simulink model "DWPT_250k_60V"  (R2026b)
settings: Solver=ode3  StopTime=0.03  FixedStep=Ts  MaxStep=1.0E-7  RelTol=1e-4  AbsTol=1e-6
model workspace (MAT data in the model file):
  CP1 = 9.99954859124e-09
  CS = 8.10569469139e-09
  CT1 = 4.27980679705e-08
  Cout = 0.00047
  Goff = 1e-08
  Ki = 20
  Kp = 0.015
  LP1 = 5e-05
  LS = 5e-05
  LT1 = 9.4696969697e-06
  M1 = 1.25e-05
  Mdesign = 1.25e-05
  RL = 30
  RP1 = 0.2
  RS = 0.2
  RT1 = 0.07
  RonSR = 0.01
  RonTx = 0.01
  Ts = 1e-08
  Vavailable = 66
  Vdc = 50
  Vtarget = 60
  averageCycles = 100
  bodyRon = 0.01
  bodyVf = 0.8
  closedLoop = 1
  deadTime = 4e-08
  f = 250000
  initialOutputVoltage = 0
  k = 0.25
  samplesPerPeriod = 400
  softStart = 0.02
  srDeadTime = 4e-08
  srEnabled = 1
  srThreshold = 0.1
  voltageHeadroom = 1.1
undefined symbols (not defined in the file or in its folder): ee_sli_rtmsupport, G, gcbh
libraries: sl_signal_attributes x63, eeGeneralControl x37, fl_lib x32, nesl_utility x28, eeGeneralMeasurement x14, ee_lib x8, dspfdesign x1
(part 2 of 3)

== system DWPT_250k_60V/Product1 ==
  Current : Inport
  Voltage : Inport  Port=2
  Average power : eeGeneralControl/Moving Average  VariantControl=Variant1  LabelModeActiveChoice=Continuous  f=f/averageCycles  x0=0  BufferSize=8192  Ts=0
      link override Continuous/Transport Delay: BufferSize=262144
  Instantaneous power : Product
  Watts : Outport
  wires:
  Current/1 -> Instantaneous power/1
  Voltage/1 -> Instantaneous power/2
  Instantaneous power/1 -> Average power/1
  Average power/1 -> Watts/1

== system DWPT_250k_60V/Product4 ==
  Current : Inport
  Voltage : Inport  Port=2
  Average power : eeGeneralControl/Moving Average  VariantControl=Variant1  LabelModeActiveChoice=Continuous  f=f/averageCycles  x0=0  BufferSize=8192  Ts=0
      link override Continuous/Transport Delay: BufferSize=262144
  Instantaneous power : Product
  Watts : Outport
  wires:
  Current/1 -> Instantaneous power/1
  Voltage/1 -> Instantaneous power/2
  Instantaneous power/1 -> Average power/1
  Average power/1 -> Watts/1

== system DWPT_250k_60V/R4 ==
  Resistor : fl_lib/Electrical/Electrical Elements/Resistor  R=RL Ohm  i_specify=off  i_priority=None  i=0 A  i_nominal_specify=off  i_nominal_value=1  i_nominal_unit=A  v_specify=off  v_priority=None  v=0 V  v_nominal_specify=off  v_nominal_value=1  v_nominal_unit=V
  + : PMIOPort  Side=Left
  - : PMIOPort  Port=2  Side=Right
  connections:
  +/RConn1 -- Resistor/LConn1
  -/RConn1 -- Resistor/RConn1

== system DWPT_250k_60V/RMS1 ==
  In : Inport
  RMS Measurement : Subsystem  LoadFcn=ee_sli_rtmsupport( 'loadfcn', gcbh );  Variant=on  VariantControlMode=label  LabelModeActiveChoice=Total  mask(RMS Measurement){F=f/averageCycles, SpecifyHarmonics=off, K=[0 1 2], InitialRMS=0, Ts=0}
      mask prompts: F "physmod:ee:library:comments:control:eeRmsMeasurement:BaseFrequencyHz_MP"; SpecifyHarmonics "physmod:ee:library:comments:control:eeRmsMeasurement:SpecifyHarmonics_MP"; K "physmod:ee:library:comments:control:eeRmsMeasurement:HarmonicNumbers_MP"; InitialRMS "physmod:ee:library:comments:control:eeRmsMeasurement:InitialRMS_MP"; Ts "physmod:ee:library:comments:control:eeGeneralControl:SampleTime1ForInherited_MP"
      mask help: physmod:ee:library:comments:control:eeRmsMeasurement:RMSMeasurement_MD
      mask init:
      | [timeDomain,G]=ee.mask.initializeRmsMeasurement(gcb,F,Ts,K,SpecifyHarmonics,InitialRMS);
      settings: CopyFcn=ee_sli_rtmsupport( 'copyfcn', gcbh );  DeleteFcn=ee_sli_rtmsupport( 'deletefcn', gcbh );  ModelCloseFcn=ee_sli_rtmsupport( 'modelclosefcn', gcbh );  PostSaveFcn=ee_sli_rtmsupport( 'postsavefcn', gcbh );  PreCopyFcn=ee_sli_rtmsupport( 'precopyfcn', gcbh );  OpenFcn=ee_sli_rtmsupport( 'openfcn', gcbh );  CloseFcn=ee_sli_rtmsupport( 'closefcn', gcbh );  PreDeleteFcn=ee_sli_rtmsupport( 'predeletefcn', gcbh );
      mask Help: web(nesl_help(gcbh))
      mask Callback SpecifyHarmonics: ee.mask.callbackRmsMeasurement(gcb);
      mask TypeOptions Ts:
      | Total RMS/Integrator
      | (Discrete or Continuous)/Ts | Total RMS/Integrator
      | (Discrete or Continuous)1/Ts | Total RMS/Periodic Difference
      | (Discrete or Continuous)/Ts | Harmonic RMS/Integrator
      | (Discrete or Continuous)/Ts | Harmonic RMS/Integrator
      | (Discrete or Continuous)1/Ts | Harmonic RMS/Periodic Difference
      | (Discrete or Continuous)/Ts | Harmonic RMS/SinCos/Integrator with
      | Wrapped State
      | (Discrete or Continuous)/Ts
      mask DialogControl F Prompt: Base frequency (Hz)
      mask DialogControl SpecifyHarmonics Prompt: Specify harmonics
      mask DialogControl K Prompt: Harmonic numbers
      mask DialogControl InitialRMS Prompt: Initial RMS
      mask DialogControl Ts Prompt: Sample time (-1 for inherited)
      mask Display: ee.mask.drawRmsMeasurement;
  RMS : Outport  VectorParamsAs1DForOutWhenUnconnected=off
  wires:
  RMS Measurement/1(RMS) -> RMS/1
  In/1 -> RMS Measurement/1(u)

== system DWPT_250k_60V/RMS10 ==
  In : Inport
  RMS Measurement : Subsystem  LoadFcn=ee_sli_rtmsupport( 'loadfcn', gcbh );  Variant=on  VariantControlMode=label  LabelModeActiveChoice=Total  mask(RMS Measurement){F=f/averageCycles, SpecifyHarmonics=off, K=[0 1 2], InitialRMS=0, Ts=0}
      mask prompts: F "physmod:ee:library:comments:control:eeRmsMeasurement:BaseFrequencyHz_MP"; SpecifyHarmonics "physmod:ee:library:comments:control:eeRmsMeasurement:SpecifyHarmonics_MP"; K "physmod:ee:library:comments:control:eeRmsMeasurement:HarmonicNumbers_MP"; InitialRMS "physmod:ee:library:comments:control:eeRmsMeasurement:InitialRMS_MP"; Ts "physmod:ee:library:comments:control:eeGeneralControl:SampleTime1ForInherited_MP"
      mask help: physmod:ee:library:comments:control:eeRmsMeasurement:RMSMeasurement_MD
      mask init:
      | [timeDomain,G]=ee.mask.initializeRmsMeasurement(gcb,F,Ts,K,SpecifyHarmonics,InitialRMS);
      settings: CopyFcn=ee_sli_rtmsupport( 'copyfcn', gcbh );  DeleteFcn=ee_sli_rtmsupport( 'deletefcn', gcbh );  ModelCloseFcn=ee_sli_rtmsupport( 'modelclosefcn', gcbh );  PostSaveFcn=ee_sli_rtmsupport( 'postsavefcn', gcbh );  PreCopyFcn=ee_sli_rtmsupport( 'precopyfcn', gcbh );  OpenFcn=ee_sli_rtmsupport( 'openfcn', gcbh );  CloseFcn=ee_sli_rtmsupport( 'closefcn', gcbh );  PreDeleteFcn=ee_sli_rtmsupport( 'predeletefcn', gcbh );
      mask Help: web(nesl_help(gcbh))
      mask Callback SpecifyHarmonics: ee.mask.callbackRmsMeasurement(gcb);
      mask TypeOptions Ts:
      | Total RMS/Integrator
      | (Discrete or Continuous)/Ts | Total RMS/Integrator
      | (Discrete or Continuous)1/Ts | Total RMS/Periodic Difference
      | (Discrete or Continuous)/Ts | Harmonic RMS/Integrator
      | (Discrete or Continuous)/Ts | Harmonic RMS/Integrator
      | (Discrete or Continuous)1/Ts | Harmonic RMS/Periodic Difference
      | (Discrete or Continuous)/Ts | Harmonic RMS/SinCos/Integrator with
      | Wrapped State
      | (Discrete or Continuous)/Ts
      mask DialogControl F Prompt: Base frequency (Hz)
      mask DialogControl SpecifyHarmonics Prompt: Specify harmonics
      mask DialogControl K Prompt: Harmonic numbers
      mask DialogControl InitialRMS Prompt: Initial RMS
      mask DialogControl Ts Prompt: Sample time (-1 for inherited)
      mask Display: ee.mask.drawRmsMeasurement;
  RMS : Outport  VectorParamsAs1DForOutWhenUnconnected=off
  wires:
  RMS Measurement/1(RMS) -> RMS/1
  In/1 -> RMS Measurement/1(u)

== system DWPT_250k_60V/RMS2 ==
  In : Inport
  RMS Measurement : Subsystem  LoadFcn=ee_sli_rtmsupport( 'loadfcn', gcbh );  Variant=on  VariantControlMode=label  LabelModeActiveChoice=Total  mask(RMS Measurement){F=f/averageCycles, SpecifyHarmonics=off, K=[0 1 2], InitialRMS=0, Ts=0}
      mask prompts: F "physmod:ee:library:comments:control:eeRmsMeasurement:BaseFrequencyHz_MP"; SpecifyHarmonics "physmod:ee:library:comments:control:eeRmsMeasurement:SpecifyHarmonics_MP"; K "physmod:ee:library:comments:control:eeRmsMeasurement:HarmonicNumbers_MP"; InitialRMS "physmod:ee:library:comments:control:eeRmsMeasurement:InitialRMS_MP"; Ts "physmod:ee:library:comments:control:eeGeneralControl:SampleTime1ForInherited_MP"
      mask help: physmod:ee:library:comments:control:eeRmsMeasurement:RMSMeasurement_MD
      mask init:
      | [timeDomain,G]=ee.mask.initializeRmsMeasurement(gcb,F,Ts,K,SpecifyHarmonics,InitialRMS);
      settings: CopyFcn=ee_sli_rtmsupport( 'copyfcn', gcbh );  DeleteFcn=ee_sli_rtmsupport( 'deletefcn', gcbh );  ModelCloseFcn=ee_sli_rtmsupport( 'modelclosefcn', gcbh );  PostSaveFcn=ee_sli_rtmsupport( 'postsavefcn', gcbh );  PreCopyFcn=ee_sli_rtmsupport( 'precopyfcn', gcbh );  OpenFcn=ee_sli_rtmsupport( 'openfcn', gcbh );  CloseFcn=ee_sli_rtmsupport( 'closefcn', gcbh );  PreDeleteFcn=ee_sli_rtmsupport( 'predeletefcn', gcbh );
      mask Help: web(nesl_help(gcbh))
      mask Callback SpecifyHarmonics: ee.mask.callbackRmsMeasurement(gcb);
      mask TypeOptions Ts:
      | Total RMS/Integrator
      | (Discrete or Continuous)/Ts | Total RMS/Integrator
      | (Discrete or Continuous)1/Ts | Total RMS/Periodic Difference
      | (Discrete or Continuous)/Ts | Harmonic RMS/Integrator
      | (Discrete or Continuous)/Ts | Harmonic RMS/Integrator
      | (Discrete or Continuous)1/Ts | Harmonic RMS/Periodic Difference
      | (Discrete or Continuous)/Ts | Harmonic RMS/SinCos/Integrator with
      | Wrapped State
      | (Discrete or Continuous)/Ts
      mask DialogControl F Prompt: Base frequency (Hz)
      mask DialogControl SpecifyHarmonics Prompt: Specify harmonics
      mask DialogControl K Prompt: Harmonic numbers
      mask DialogControl InitialRMS Prompt: Initial RMS
      mask DialogControl Ts Prompt: Sample time (-1 for inherited)
      mask Display: ee.mask.drawRmsMeasurement;
  RMS : Outport  VectorParamsAs1DForOutWhenUnconnected=off
  wires:
  RMS Measurement/1(RMS) -> RMS/1
  In/1 -> RMS Measurement/1(u)

== system DWPT_250k_60V/RMS3 ==
  In : Inport
  RMS Measurement : Subsystem  LoadFcn=ee_sli_rtmsupport( 'loadfcn', gcbh );  Variant=on  VariantControlMode=label  LabelModeActiveChoice=Total  mask(RMS Measurement){F=f/averageCycles, SpecifyHarmonics=off, K=[0 1 2], InitialRMS=0, Ts=0}
      mask prompts: F "physmod:ee:library:comments:control:eeRmsMeasurement:BaseFrequencyHz_MP"; SpecifyHarmonics "physmod:ee:library:comments:control:eeRmsMeasurement:SpecifyHarmonics_MP"; K "physmod:ee:library:comments:control:eeRmsMeasurement:HarmonicNumbers_MP"; InitialRMS "physmod:ee:library:comments:control:eeRmsMeasurement:InitialRMS_MP"; Ts "physmod:ee:library:comments:control:eeGeneralControl:SampleTime1ForInherited_MP"
      mask help: physmod:ee:library:comments:control:eeRmsMeasurement:RMSMeasurement_MD
      mask init:
      | [timeDomain,G]=ee.mask.initializeRmsMeasurement(gcb,F,Ts,K,SpecifyHarmonics,InitialRMS);
      settings: CopyFcn=ee_sli_rtmsupport( 'copyfcn', gcbh );  DeleteFcn=ee_sli_rtmsupport( 'deletefcn', gcbh );  ModelCloseFcn=ee_sli_rtmsupport( 'modelclosefcn', gcbh );  PostSaveFcn=ee_sli_rtmsupport( 'postsavefcn', gcbh );  PreCopyFcn=ee_sli_rtmsupport( 'precopyfcn', gcbh );  OpenFcn=ee_sli_rtmsupport( 'openfcn', gcbh );  CloseFcn=ee_sli_rtmsupport( 'closefcn', gcbh );  PreDeleteFcn=ee_sli_rtmsupport( 'predeletefcn', gcbh );
      mask Help: web(nesl_help(gcbh))
      mask Callback SpecifyHarmonics: ee.mask.callbackRmsMeasurement(gcb);
      mask TypeOptions Ts:
      | Total RMS/Integrator
      | (Discrete or Continuous)/Ts | Total RMS/Integrator
      | (Discrete or Continuous)1/Ts | Total RMS/Periodic Difference
      | (Discrete or Continuous)/Ts | Harmonic RMS/Integrator
      | (Discrete or Continuous)/Ts | Harmonic RMS/Integrator
      | (Discrete or Continuous)1/Ts | Harmonic RMS/Periodic Difference
      | (Discrete or Continuous)/Ts | Harmonic RMS/SinCos/Integrator with
      | Wrapped State
      | (Discrete or Continuous)/Ts
      mask DialogControl F Prompt: Base frequency (Hz)
      mask DialogControl SpecifyHarmonics Prompt: Specify harmonics
      mask DialogControl K Prompt: Harmonic numbers
      mask DialogControl InitialRMS Prompt: Initial RMS
      mask DialogControl Ts Prompt: Sample time (-1 for inherited)
      mask Display: ee.mask.drawRmsMeasurement;
  RMS : Outport  VectorParamsAs1DForOutWhenUnconnected=off
  wires:
  RMS Measurement/1(RMS) -> RMS/1
  In/1 -> RMS Measurement/1(u)

== system DWPT_250k_60V/RMS4 ==
  In : Inport
  RMS Measurement : Subsystem  LoadFcn=ee_sli_rtmsupport( 'loadfcn', gcbh );  Variant=on  VariantControlMode=label  LabelModeActiveChoice=Total  mask(RMS Measurement){F=f/averageCycles, SpecifyHarmonics=off, K=[0 1 2], InitialRMS=0, Ts=0}
      mask prompts: F "physmod:ee:library:comments:control:eeRmsMeasurement:BaseFrequencyHz_MP"; SpecifyHarmonics "physmod:ee:library:comments:control:eeRmsMeasurement:SpecifyHarmonics_MP"; K "physmod:ee:library:comments:control:eeRmsMeasurement:HarmonicNumbers_MP"; InitialRMS "physmod:ee:library:comments:control:eeRmsMeasurement:InitialRMS_MP"; Ts "physmod:ee:library:comments:control:eeGeneralControl:SampleTime1ForInherited_MP"
      mask help: physmod:ee:library:comments:control:eeRmsMeasurement:RMSMeasurement_MD
      mask init:
      | [timeDomain,G]=ee.mask.initializeRmsMeasurement(gcb,F,Ts,K,SpecifyHarmonics,InitialRMS);
      settings: CopyFcn=ee_sli_rtmsupport( 'copyfcn', gcbh );  DeleteFcn=ee_sli_rtmsupport( 'deletefcn', gcbh );  ModelCloseFcn=ee_sli_rtmsupport( 'modelclosefcn', gcbh );  PostSaveFcn=ee_sli_rtmsupport( 'postsavefcn', gcbh );  PreCopyFcn=ee_sli_rtmsupport( 'precopyfcn', gcbh );  OpenFcn=ee_sli_rtmsupport( 'openfcn', gcbh );  CloseFcn=ee_sli_rtmsupport( 'closefcn', gcbh );  PreDeleteFcn=ee_sli_rtmsupport( 'predeletefcn', gcbh );
      mask Help: web(nesl_help(gcbh))
      mask Callback SpecifyHarmonics: ee.mask.callbackRmsMeasurement(gcb);
      mask TypeOptions Ts:
      | Total RMS/Integrator
      | (Discrete or Continuous)/Ts | Total RMS/Integrator
      | (Discrete or Continuous)1/Ts | Total RMS/Periodic Difference
      | (Discrete or Continuous)/Ts | Harmonic RMS/Integrator
      | (Discrete or Continuous)/Ts | Harmonic RMS/Integrator
      | (Discrete or Continuous)1/Ts | Harmonic RMS/Periodic Difference
      | (Discrete or Continuous)/Ts | Harmonic RMS/SinCos/Integrator with
      | Wrapped State
      | (Discrete or Continuous)/Ts
      mask DialogControl F Prompt: Base frequency (Hz)
      mask DialogControl SpecifyHarmonics Prompt: Specify harmonics
      mask DialogControl K Prompt: Harmonic numbers
      mask DialogControl InitialRMS Prompt: Initial RMS
      mask DialogControl Ts Prompt: Sample time (-1 for inherited)
      mask Display: ee.mask.drawRmsMeasurement;
  RMS : Outport  VectorParamsAs1DForOutWhenUnconnected=off
  wires:
  RMS Measurement/1(RMS) -> RMS/1
  In/1 -> RMS Measurement/1(u)

== system DWPT_250k_60V/RMS6 ==
  In : Inport
  RMS Measurement : Subsystem  LoadFcn=ee_sli_rtmsupport( 'loadfcn', gcbh );  Variant=on  VariantControlMode=label  LabelModeActiveChoice=Total  mask(RMS Measurement){F=f/averageCycles, SpecifyHarmonics=off, K=[0 1 2], InitialRMS=0, Ts=0}
      mask prompts: F "physmod:ee:library:comments:control:eeRmsMeasurement:BaseFrequencyHz_MP"; SpecifyHarmonics "physmod:ee:library:comments:control:eeRmsMeasurement:SpecifyHarmonics_MP"; K "physmod:ee:library:comments:control:eeRmsMeasurement:HarmonicNumbers_MP"; InitialRMS "physmod:ee:library:comments:control:eeRmsMeasurement:InitialRMS_MP"; Ts "physmod:ee:library:comments:control:eeGeneralControl:SampleTime1ForInherited_MP"
      mask help: physmod:ee:library:comments:control:eeRmsMeasurement:RMSMeasurement_MD
      mask init:
      | [timeDomain,G]=ee.mask.initializeRmsMeasurement(gcb,F,Ts,K,SpecifyHarmonics,InitialRMS);
      settings: CopyFcn=ee_sli_rtmsupport( 'copyfcn', gcbh );  DeleteFcn=ee_sli_rtmsupport( 'deletefcn', gcbh );  ModelCloseFcn=ee_sli_rtmsupport( 'modelclosefcn', gcbh );  PostSaveFcn=ee_sli_rtmsupport( 'postsavefcn', gcbh );  PreCopyFcn=ee_sli_rtmsupport( 'precopyfcn', gcbh );  OpenFcn=ee_sli_rtmsupport( 'openfcn', gcbh );  CloseFcn=ee_sli_rtmsupport( 'closefcn', gcbh );  PreDeleteFcn=ee_sli_rtmsupport( 'predeletefcn', gcbh );
      mask Help: web(nesl_help(gcbh))
      mask Callback SpecifyHarmonics: ee.mask.callbackRmsMeasurement(gcb);
      mask TypeOptions Ts:
      | Total RMS/Integrator
      | (Discrete or Continuous)/Ts | Total RMS/Integrator
      | (Discrete or Continuous)1/Ts | Total RMS/Periodic Difference
      | (Discrete or Continuous)/Ts | Harmonic RMS/Integrator
      | (Discrete or Continuous)/Ts | Harmonic RMS/Integrator
      | (Discrete or Continuous)1/Ts | Harmonic RMS/Periodic Difference
      | (Discrete or Continuous)/Ts | Harmonic RMS/SinCos/Integrator with
      | Wrapped State
      | (Discrete or Continuous)/Ts
      mask DialogControl F Prompt: Base frequency (Hz)
      mask DialogControl SpecifyHarmonics Prompt: Specify harmonics
      mask DialogControl K Prompt: Harmonic numbers
      mask DialogControl InitialRMS Prompt: Initial RMS
      mask DialogControl Ts Prompt: Sample time (-1 for inherited)
      mask Display: ee.mask.drawRmsMeasurement;
  RMS : Outport  VectorParamsAs1DForOutWhenUnconnected=off
  wires:
  RMS Measurement/1(RMS) -> RMS/1
  In/1 -> RMS Measurement/1(u)

== system DWPT_250k_60V/RMS8 ==
  In : Inport
  RMS Measurement : Subsystem  LoadFcn=ee_sli_rtmsupport( 'loadfcn', gcbh );  Variant=on  VariantControlMode=label  LabelModeActiveChoice=Total  mask(RMS Measurement){F=f/averageCycles, SpecifyHarmonics=off, K=[0 1 2], InitialRMS=0, Ts=0}
      mask prompts: F "physmod:ee:library:comments:control:eeRmsMeasurement:BaseFrequencyHz_MP"; SpecifyHarmonics "physmod:ee:library:comments:control:eeRmsMeasurement:SpecifyHarmonics_MP"; K "physmod:ee:library:comments:control:eeRmsMeasurement:HarmonicNumbers_MP"; InitialRMS "physmod:ee:library:comments:control:eeRmsMeasurement:InitialRMS_MP"; Ts "physmod:ee:library:comments:control:eeGeneralControl:SampleTime1ForInherited_MP"
      mask help: physmod:ee:library:comments:control:eeRmsMeasurement:RMSMeasurement_MD
      mask init:
      | [timeDomain,G]=ee.mask.initializeRmsMeasurement(gcb,F,Ts,K,SpecifyHarmonics,InitialRMS);
      settings: CopyFcn=ee_sli_rtmsupport( 'copyfcn', gcbh );  DeleteFcn=ee_sli_rtmsupport( 'deletefcn', gcbh );  ModelCloseFcn=ee_sli_rtmsupport( 'modelclosefcn', gcbh );  PostSaveFcn=ee_sli_rtmsupport( 'postsavefcn', gcbh );  PreCopyFcn=ee_sli_rtmsupport( 'precopyfcn', gcbh );  OpenFcn=ee_sli_rtmsupport( 'openfcn', gcbh );  CloseFcn=ee_sli_rtmsupport( 'closefcn', gcbh );  PreDeleteFcn=ee_sli_rtmsupport( 'predeletefcn', gcbh );
      mask Help: web(nesl_help(gcbh))
      mask Callback SpecifyHarmonics: ee.mask.callbackRmsMeasurement(gcb);
      mask TypeOptions Ts:
      | Total RMS/Integrator
      | (Discrete or Continuous)/Ts | Total RMS/Integrator
      | (Discrete or Continuous)1/Ts | Total RMS/Periodic Difference
      | (Discrete or Continuous)/Ts | Harmonic RMS/Integrator
      | (Discrete or Continuous)/Ts | Harmonic RMS/Integrator
      | (Discrete or Continuous)1/Ts | Harmonic RMS/Periodic Difference
      | (Discrete or Continuous)/Ts | Harmonic RMS/SinCos/Integrator with
      | Wrapped State
      | (Discrete or Continuous)/Ts
      mask DialogControl F Prompt: Base frequency (Hz)
      mask DialogControl SpecifyHarmonics Prompt: Specify harmonics
      mask DialogControl K Prompt: Harmonic numbers
      mask DialogControl InitialRMS Prompt: Initial RMS
      mask DialogControl Ts Prompt: Sample time (-1 for inherited)
      mask Display: ee.mask.drawRmsMeasurement;
  RMS : Outport  VectorParamsAs1DForOutWhenUnconnected=off
  wires:
  RMS Measurement/1(RMS) -> RMS/1
  In/1 -> RMS Measurement/1(u)

== system DWPT_250k_60V/RX coil voltage ==
  PS-Simulink Converter : nesl_utility/PS-Simulink Converter  PhysicalDomain=network_engine_domain  SubClassName=ps_output  LeftPortType=input  RightPortType=output  PseudoPeriodic=off  Frequencies=[]  VectorFormat=1-D array  Unit=V  AffineConversion=off
  Voltage Sensor : fl_lib/Electrical/Electrical Sensors/Voltage Sensor
  + : PMIOPort  Side=Left
  - : PMIOPort  Port=2  Side=Left
  v : Outport  VectorParamsAs1DForOutWhenUnconnected=off
  wires:
  PS-Simulink Converter/1 -> v/1
  connections:
  +/RConn1 -- Voltage Sensor/LConn1
  -/RConn1 -- Voltage Sensor/RConn2
  PS-Simulink Converter/LConn1 -- Voltage Sensor/RConn1

== system DWPT_250k_60V/Rectifier DC current ==
  Current Sensor : fl_lib/Electrical/Electrical Sensors/Current Sensor
  PS-Simulink Converter : nesl_utility/PS-Simulink Converter  PhysicalDomain=network_engine_domain  SubClassName=ps_output  LeftPortType=input  RightPortType=output  PseudoPeriodic=off  Frequencies=[]  VectorFormat=1-D array  Unit=A  AffineConversion=off
  + : PMIOPort  Side=Left
  - : PMIOPort  Port=2  Side=Right
  i : Outport  VectorParamsAs1DForOutWhenUnconnected=off
  wires:
  PS-Simulink Converter/1 -> i/1
  connections:
  PS-Simulink Converter/LConn1 -- Current Sensor/RConn1
  -/RConn1 -- Current Sensor/RConn2
  +/RConn1 -- Current Sensor/LConn1

== system DWPT_250k_60V/Synchronous Rectifier ==
  Positive current gates : Inport
  Negative current gates : Inport  Port=2
  Q1 : Subsystem
  Q2 : Subsystem
  Q3 : Subsystem
  Q4 : Subsystem
  AC A : PMIOPort  Side=Left
  AC B : PMIOPort  Port=2  Side=Left
  DC plus : PMIOPort  Port=3  Side=Right
  DC minus : PMIOPort  Port=4  Side=Right
  wires:
  Positive current gates/1 -> Q1/1(g), Q4/1(g)
  Negative current gates/1 -> Q2/1(g), Q3/1(g)
  connections:
  Q1/LConn1 -- DC plus/RConn1 -- Q2/LConn1
  Q1/RConn1 -- AC A/RConn1 -- Q3/LConn1
  Q2/RConn1 -- AC B/RConn1 -- Q4/LConn1
  Q3/RConn1 -- DC minus/RConn1 -- Q4/RConn1

== system DWPT_250k_60V/TX coil current ==
  Current Sensor : fl_lib/Electrical/Electrical Sensors/Current Sensor
  PS-Simulink Converter : nesl_utility/PS-Simulink Converter  PhysicalDomain=network_engine_domain  SubClassName=ps_output  LeftPortType=input  RightPortType=output  PseudoPeriodic=off  Frequencies=[]  VectorFormat=1-D array  Unit=A  AffineConversion=off
  + : PMIOPort  Side=Left
  - : PMIOPort  Port=2  Side=Right
  i : Outport  VectorParamsAs1DForOutWhenUnconnected=off
  wires:
  PS-Simulink Converter/1 -> i/1
  connections:
  PS-Simulink Converter/LConn1 -- Current Sensor/RConn1
  -/RConn1 -- Current Sensor/RConn2
  +/RConn1 -- Current Sensor/LConn1

== system DWPT_250k_60V/TX coil voltage ==
  PS-Simulink Converter : nesl_utility/PS-Simulink Converter  PhysicalDomain=network_engine_domain  SubClassName=ps_output  LeftPortType=input  RightPortType=output  PseudoPeriodic=off  Frequencies=[]  VectorFormat=1-D array  Unit=V  AffineConversion=off
  Voltage Sensor : fl_lib/Electrical/Electrical Sensors/Voltage Sensor
  + : PMIOPort  Side=Left
  - : PMIOPort  Port=2  Side=Left
  v : Outport  VectorParamsAs1DForOutWhenUnconnected=off
  wires:
  PS-Simulink Converter/1 -> v/1
  connections:
  +/RConn1 -- Voltage Sensor/LConn1
  -/RConn1 -- Voltage Sensor/RConn2
  PS-Simulink Converter/LConn1 -- Voltage Sensor/RConn1

== system DWPT_250k_60V/Uo2 ==
  PS-Simulink Converter : nesl_utility/PS-Simulink Converter  PhysicalDomain=network_engine_domain  SubClassName=ps_output  LeftPortType=input  RightPortType=output  PseudoPeriodic=off  Frequencies=[]  VectorFormat=1-D array  Unit=V  AffineConversion=off
  Voltage Sensor : fl_lib/Electrical/Electrical Sensors/Voltage Sensor
  + : PMIOPort  Side=Left
  - : PMIOPort  Port=2  Side=Left
  v : Outport  VectorParamsAs1DForOutWhenUnconnected=off
  wires:
  PS-Simulink Converter/1 -> v/1
  connections:
  PS-Simulink Converter/LConn1 -- Voltage Sensor/RConn1
  -/RConn1 -- Voltage Sensor/RConn2
  +/RConn1 -- Voltage Sensor/LConn1

== system DWPT_250k_60V/V M ==
  PS-Simulink Converter : nesl_utility/PS-Simulink Converter  PhysicalDomain=network_engine_domain  SubClassName=ps_output  LeftPortType=input  RightPortType=output  PseudoPeriodic=off  Frequencies=[]  VectorFormat=1-D array  Unit=V  AffineConversion=off
  Voltage Sensor : fl_lib/Electrical/Electrical Sensors/Voltage Sensor
  + : PMIOPort  Side=Left
  - : PMIOPort  Port=2  Side=Left
  v : Outport  VectorParamsAs1DForOutWhenUnconnected=off
  wires:
  PS-Simulink Converter/1 -> v/1
  connections:
  PS-Simulink Converter/LConn1 -- Voltage Sensor/RConn1
  -/RConn1 -- Voltage Sensor/RConn2
  +/RConn1 -- Voltage Sensor/LConn1

== system DWPT_250k_60V/V M1 ==
  PS-Simulink Converter : nesl_utility/PS-Simulink Converter  PhysicalDomain=network_engine_domain  SubClassName=ps_output  LeftPortType=input  RightPortType=output  PseudoPeriodic=off  Frequencies=[]  VectorFormat=1-D array  Unit=V  AffineConversion=off
  Voltage Sensor : fl_lib/Electrical/Electrical Sensors/Voltage Sensor
  + : PMIOPort  Side=Left
  - : PMIOPort  Port=2  Side=Left
  v : Outport  VectorParamsAs1DForOutWhenUnconnected=off
  wires:
  PS-Simulink Converter/1 -> v/1
  connections:
  PS-Simulink Converter/LConn1 -- Voltage Sensor/RConn1
  -/RConn1 -- Voltage Sensor/RConn2
  +/RConn1 -- Voltage Sensor/LConn1

== system DWPT_250k_60V/V M3 ==
  PS-Simulink Converter : nesl_utility/PS-Simulink Converter  PhysicalDomain=network_engine_domain  SubClassName=ps_output  LeftPortType=input  RightPortType=output  PseudoPeriodic=off  Frequencies=[]  VectorFormat=1-D array  Unit=V  AffineConversion=off
  Voltage Sensor : fl_lib/Electrical/Electrical Sensors/Voltage Sensor
  + : PMIOPort  Side=Left
  - : PMIOPort  Port=2  Side=Left
  v : Outport  VectorParamsAs1DForOutWhenUnconnected=off
  wires:
  PS-Simulink Converter/1 -> v/1
  connections:
  PS-Simulink Converter/LConn1 -- Voltage Sensor/RConn1
  -/RConn1 -- Voltage Sensor/RConn2
  +/RConn1 -- Voltage Sensor/LConn1

== system DWPT_250k_60V/V M5 ==
  PS-Simulink Converter : nesl_utility/PS-Simulink Converter  PhysicalDomain=network_engine_domain  SubClassName=ps_output  LeftPortType=input  RightPortType=output  PseudoPeriodic=off  Frequencies=[]  VectorFormat=1-D array  Unit=V  AffineConversion=off
  Voltage Sensor : fl_lib/Electrical/Electrical Sensors/Voltage Sensor
  + : PMIOPort  Side=Left
  - : PMIOPort  Port=2  Side=Left
  v : Outport  VectorParamsAs1DForOutWhenUnconnected=off
  wires:
  PS-Simulink Converter/1 -> v/1
  connections:
  PS-Simulink Converter/LConn1 -- Voltage Sensor/RConn1
  -/RConn1 -- Voltage Sensor/RConn2
  +/RConn1 -- Voltage Sensor/LConn1

== system DWPT_250k_60V/RMS1/RMS Measurement ==
  u : Inport
  Harmonic RMS : Subsystem  VariantControl=Harmonic
  Total RMS : Subsystem  VariantControl=Total
  RMS : Outport  VectorParamsAs1DForOutWhenUnconnected=off

== system DWPT_250k_60V/RMS10/RMS Measurement ==
  u : Inport
  Harmonic RMS : Subsystem  VariantControl=Harmonic
  Total RMS : Subsystem  VariantControl=Total
  RMS : Outport  VectorParamsAs1DForOutWhenUnconnected=off

== system DWPT_250k_60V/RMS2/RMS Measurement ==
  u : Inport
  Harmonic RMS : Subsystem  VariantControl=Harmonic
  Total RMS : Subsystem  VariantControl=Total
  RMS : Outport  VectorParamsAs1DForOutWhenUnconnected=off

== system DWPT_250k_60V/RMS3/RMS Measurement ==
  u : Inport
  Harmonic RMS : Subsystem  VariantControl=Harmonic
  Total RMS : Subsystem  VariantControl=Total
  RMS : Outport  VectorParamsAs1DForOutWhenUnconnected=off

== system DWPT_250k_60V/RMS4/RMS Measurement ==
  u : Inport
  Harmonic RMS : Subsystem  VariantControl=Harmonic
  Total RMS : Subsystem  VariantControl=Total
  RMS : Outport  VectorParamsAs1DForOutWhenUnconnected=off

== system DWPT_250k_60V/RMS6/RMS Measurement ==
  u : Inport
  Harmonic RMS : Subsystem  VariantControl=Harmonic
  Total RMS : Subsystem  VariantControl=Total
  RMS : Outport  VectorParamsAs1DForOutWhenUnconnected=off

== system DWPT_250k_60V/RMS8/RMS Measurement ==
  u : Inport
  Harmonic RMS : Subsystem  VariantControl=Harmonic
  Total RMS : Subsystem  VariantControl=Total
  RMS : Outport  VectorParamsAs1DForOutWhenUnconnected=off

== system DWPT_250k_60V/Synchronous Rectifier/Q1 ==
  g : Inport
  Data Type Conversion : DataTypeConversion  OutDataTypeStr=double  SaturateOnIntegerOverflow=off  RndMeth=Floor
  MOSFET : ee_lib/Semiconductors & Converters/MOSFET (Ideal, Switching)  port_option=ee.enum.controlport.ps  Rds=RonSR Ohm  Goff=Goff 1/Ohm  Vth=0.5 V  diode_param=2  diode_Vf=bodyVf V  diode_Ron=bodyRon Ohm  diode_Goff=Goff 1/Ohm  diode_C=5e-8 F  diode_iRM=-235 A  diode_iF=300 A  diode_idot=-50 A/us  diode_trr_param=1  diode_trr_factor=3  diode_trr=15 us  diode_Qrr=1.5e+3 s*uA  ids_specify=off  ids_priority=None  ids=0 A  ids_nominal_specify=off  ids_nominal_value=1  ids_nominal_unit=A  vds_specify=off  vds_priority=None  vds=0 V  vds_nominal_specify=off  vds_nominal_value=1  vds_nominal_unit=V  vgs_specify=off  vgs_priority=None  vgs=0 V  vgs_nominal_specify=off  vgs_nominal_value=1  vgs_nominal_unit=V  thermal_loss_option=ee.enum.converters.thermalLossOption.constantvalues  Von_data=[0, 1.1, 1.3, 1.45, 1.75, 2.25, 2.7; 0, 1, 1.15, 1.35, 1.7, 2.35, 3] V  Tj=[298.15, 398.15] K  Iout_data=[0, 10, 50, 100, 200, 400, 600] A  tabulateWithVds=false  Eon_data=[0, .29, 1.43, 2.86, 5.71, 13.14, 22.86; 0, .57, 2.63, 5.14, 10.29, 20.57, 30.29] * 1e-3 J  Eoff_data=[0, .21, 1.07, 2.14, 4.29, 9.86, 17.14; 0, .43, 1.97, 3.86, 7.71, 15.43, 22.71] * 1e-3 J  Eon_data_3D=[zeros(2, 5, 3)] J  Eoff_data_3D=[zeros(2, 5, 3)] J  Tj_loss=[298.15, 448.15] K  Iout_data_loss=[0, 10, 20, 30, 40] A  Vds_loss=[0, 150, 300] V  Eon_scalar=22.86e-3 J  Eoff_scalar=17.14e-3 J  Voff=300 V  Iout_scalar=600 A  useCurrentFromPreviousCycle=true  currentMeasDelay=0 s  useVoltageFromPreviousCycle=true  voltageMeasDelay=0 s  diodeModelType=ee.enum.converters.diodeModelType.pwl  diodeTableType=ee.enum.diode.tableType.IfMat  diode_ReverseIVType=ee.enum.diode.diodeReverseIV.constant  diode_IfMat=[.07, .12, .19, 1.75, 4.24, 7.32, 11.2; .16, .3, .72, 2.14, 4.02, 6.35, 9.12] A  diode_VfMat=[.9, 1.15, 1.25, 1.5, 1.75, 2.17, 2.6, 2.85; .58, .68, .75, 1.1, 1.38, 1.77, 2.27, 2.7] V  diode_TjVec=[25, 125] degC  diode_VfVec=[.5, .7, .9, 1.3, 1.7, 2.1, 2.5] V  diode_IfVec=[.1, .2, .5, 1, 2, 4, 7, 10] A  diode_IrMat=[1e-06, 2e-06, 5e-06, 1e-05, 2.5e-05, 5e-05, .0001; 2e-06, 5e-06, 1e-05, 4e-05, 8e-05, .0002, .0005] A  diode_VrMat=[10, 100, 200, 250, 300, 325, 350; 10, 70, 160, 220, 270, 300, 320] V  diode_VrVec=[10, 20, 40, 50, 70, 80, 100] V  diode_IrVec=[1e-06, 2e-06, 5e-06, 1e-05, 2e-05, 5e-05, .0001] A  diode_Vr=-600 V  diode_Ls=150 nH  diode_Erec=0.03 J  diode_rec_loss_model=ee.enum.diode.reverseRecoveryModelTabulateUpTo3D.fixed  diode_ErecVal=0 J  diode_scaleWithIandV=true  diode_ErecMat=zeros(2, 3) J  diodeErecMat3D=zeros(2, 3, 2) J  diode_TjrecVec=[298.15, 398.15] K  diode_IfrecVec=[.1, 1, 10] A  diodeVrecVec=[0, 100] V  diode_IrecVal=10 A  diode_VrecVal=10 V  diode_tFilter=1 / 1000 / 100 s  separateThermalPortForDiode=false  thermal_network_parameterization=ee.enum.thermalNetworkTopology.external  Rth=[.03, .2] K/W  Rth_Cauer=[.03, .1, .2] K/W  Rth_Foster=[.03, .2] K/W  thermal_mass_parameterization=ee.enum.thermalNetwork.timeconstant  thermal_mass=[3, 25] J/K  thermal_mass_Cauer=[3, 10, 25] J/K  thermal_mass_Foster=[33, 50] J/K  thermal_time_constant=[.1, 5] s  thermal_time_constant_Cauer=[.1, 1, 5] s  thermal_time_constant_Foster=[1, 10] s  thermal_mass_initial_temperatures=[25, 25] degC  thermal_mass_initial_temperatures_Cauer=[25, 25, 25] degC  junction_thermal_mass=0.1 J/K  Tvec_initial_Foster=[25, 25, 25, 25] degC  RthDiode=[.03, .2] K/W  RthCauerDiode=[.03, .1, .2] K/W  RthFosterDiode=[.03, .2] K/W  thermalMassDiode=[3, 25] J/K  thermalMassCauerDiode=[3, 10, 25] J/K  thermalMassFosterDiode=[33, 50] J/K  thermalTauDiode=[.1, 5] s  thermalTauCauerDiode=[.1, 1, 5] s  thermalTauFosterDiode=[1, 10] s  thermalMassInitTempDiode=[25, 25] degC  thermalMassInitTempCauerDiode=[25, 25, 25] degC  junctionthermalMassDiode=0.1 J/K  TVecInitialFosterDiode=[25, 25] degC  no_thermal_network=ee.enum.enable.no  mosfet_junction_temperature_specify=off  mosfet_junction_temperature_priority=None  mosfet_junction_temperature=25 degC  mosfet_junction_temperature_nominal_specify=off  mosfet_junction_temperature_nominal_value=1  mosfet_junction_temperature_nominal_unit=degC  diode_junction_temperature_specify=off  diode_junction_temperature_priority=None  diode_junction_temperature=25 degC  diode_junction_temperature_nominal_specify=off  diode_junction_temperature_nominal_value=1  diode_junction_temperature_nominal_unit=degC  Qj_specify=off  Qj_priority=None  Qj=0 W  Qj_nominal_specify=off  Qj_nominal_value=1  Qj_nominal_unit=W  accumulatedSwitchingLosses_specify=off  accumulatedSwitchingLosses_priority=None  accumulatedSwitchingLosses=0 J
  Simulink-PS Converter : nesl_utility/Simulink-PS Converter  PhysicalDomain=network_engine_domain  SubClassName=ps_input  LeftPortType=input  RightPortType=output  PseudoPeriodic=off  Frequencies=[]  NoiseDistribution=none  NoiseParameters=[]  Unit=1  AffineConversion=off  FilteringAndDerivatives=provide  SimscapeFilterOrder=1  InputFilterTimeConstant=0.001  UdotUserProvided=0
  D : PMIOPort  Side=Left
  S : PMIOPort  Port=2  Side=Right
  wires:
  Data Type Conversion/1 -> Simulink-PS Converter/1
  g/1 -> Data Type Conversion/1
  connections:
  MOSFET/RConn1 -- D/RConn1
  Simulink-PS Converter/RConn1 -- MOSFET/LConn1
  S/RConn1 -- MOSFET/RConn2

== system DWPT_250k_60V/Synchronous Rectifier/Q2 ==
  g : Inport
  Data Type Conversion : DataTypeConversion  OutDataTypeStr=double  SaturateOnIntegerOverflow=off  RndMeth=Floor
  MOSFET : ee_lib/Semiconductors & Converters/MOSFET (Ideal, Switching)  port_option=ee.enum.controlport.ps  Rds=RonSR Ohm  Goff=Goff 1/Ohm  Vth=0.5 V  diode_param=2  diode_Vf=bodyVf V  diode_Ron=bodyRon Ohm  diode_Goff=Goff 1/Ohm  diode_C=5e-8 F  diode_iRM=-235 A  diode_iF=300 A  diode_idot=-50 A/us  diode_trr_param=1  diode_trr_factor=3  diode_trr=15 us  diode_Qrr=1.5e+3 s*uA  ids_specify=off  ids_priority=None  ids=0 A  ids_nominal_specify=off  ids_nominal_value=1  ids_nominal_unit=A  vds_specify=off  vds_priority=None  vds=0 V  vds_nominal_specify=off  vds_nominal_value=1  vds_nominal_unit=V  vgs_specify=off  vgs_priority=None  vgs=0 V  vgs_nominal_specify=off  vgs_nominal_value=1  vgs_nominal_unit=V  thermal_loss_option=ee.enum.converters.thermalLossOption.constantvalues  Von_data=[0, 1.1, 1.3, 1.45, 1.75, 2.25, 2.7; 0, 1, 1.15, 1.35, 1.7, 2.35, 3] V  Tj=[298.15, 398.15] K  Iout_data=[0, 10, 50, 100, 200, 400, 600] A  tabulateWithVds=false  Eon_data=[0, .29, 1.43, 2.86, 5.71, 13.14, 22.86; 0, .57, 2.63, 5.14, 10.29, 20.57, 30.29] * 1e-3 J  Eoff_data=[0, .21, 1.07, 2.14, 4.29, 9.86, 17.14; 0, .43, 1.97, 3.86, 7.71, 15.43, 22.71] * 1e-3 J  Eon_data_3D=[zeros(2, 5, 3)] J  Eoff_data_3D=[zeros(2, 5, 3)] J  Tj_loss=[298.15, 448.15] K  Iout_data_loss=[0, 10, 20, 30, 40] A  Vds_loss=[0, 150, 300] V  Eon_scalar=22.86e-3 J  Eoff_scalar=17.14e-3 J  Voff=300 V  Iout_scalar=600 A  useCurrentFromPreviousCycle=true  currentMeasDelay=0 s  useVoltageFromPreviousCycle=true  voltageMeasDelay=0 s  diodeModelType=ee.enum.converters.diodeModelType.pwl  diodeTableType=ee.enum.diode.tableType.IfMat  diode_ReverseIVType=ee.enum.diode.diodeReverseIV.constant  diode_IfMat=[.07, .12, .19, 1.75, 4.24, 7.32, 11.2; .16, .3, .72, 2.14, 4.02, 6.35, 9.12] A  diode_VfMat=[.9, 1.15, 1.25, 1.5, 1.75, 2.17, 2.6, 2.85; .58, .68, .75, 1.1, 1.38, 1.77, 2.27, 2.7] V  diode_TjVec=[25, 125] degC  diode_VfVec=[.5, .7, .9, 1.3, 1.7, 2.1, 2.5] V  diode_IfVec=[.1, .2, .5, 1, 2, 4, 7, 10] A  diode_IrMat=[1e-06, 2e-06, 5e-06, 1e-05, 2.5e-05, 5e-05, .0001; 2e-06, 5e-06, 1e-05, 4e-05, 8e-05, .0002, .0005] A  diode_VrMat=[10, 100, 200, 250, 300, 325, 350; 10, 70, 160, 220, 270, 300, 320] V  diode_VrVec=[10, 20, 40, 50, 70, 80, 100] V  diode_IrVec=[1e-06, 2e-06, 5e-06, 1e-05, 2e-05, 5e-05, .0001] A  diode_Vr=-600 V  diode_Ls=150 nH  diode_Erec=0.03 J  diode_rec_loss_model=ee.enum.diode.reverseRecoveryModelTabulateUpTo3D.fixed  diode_ErecVal=0 J  diode_scaleWithIandV=true  diode_ErecMat=zeros(2, 3) J  diodeErecMat3D=zeros(2, 3, 2) J  diode_TjrecVec=[298.15, 398.15] K  diode_IfrecVec=[.1, 1, 10] A  diodeVrecVec=[0, 100] V  diode_IrecVal=10 A  diode_VrecVal=10 V  diode_tFilter=1 / 1000 / 100 s  separateThermalPortForDiode=false  thermal_network_parameterization=ee.enum.thermalNetworkTopology.external  Rth=[.03, .2] K/W  Rth_Cauer=[.03, .1, .2] K/W  Rth_Foster=[.03, .2] K/W  thermal_mass_parameterization=ee.enum.thermalNetwork.timeconstant  thermal_mass=[3, 25] J/K  thermal_mass_Cauer=[3, 10, 25] J/K  thermal_mass_Foster=[33, 50] J/K  thermal_time_constant=[.1, 5] s  thermal_time_constant_Cauer=[.1, 1, 5] s  thermal_time_constant_Foster=[1, 10] s  thermal_mass_initial_temperatures=[25, 25] degC  thermal_mass_initial_temperatures_Cauer=[25, 25, 25] degC  junction_thermal_mass=0.1 J/K  Tvec_initial_Foster=[25, 25, 25, 25] degC  RthDiode=[.03, .2] K/W  RthCauerDiode=[.03, .1, .2] K/W  RthFosterDiode=[.03, .2] K/W  thermalMassDiode=[3, 25] J/K  thermalMassCauerDiode=[3, 10, 25] J/K  thermalMassFosterDiode=[33, 50] J/K  thermalTauDiode=[.1, 5] s  thermalTauCauerDiode=[.1, 1, 5] s  thermalTauFosterDiode=[1, 10] s  thermalMassInitTempDiode=[25, 25] degC  thermalMassInitTempCauerDiode=[25, 25, 25] degC  junctionthermalMassDiode=0.1 J/K  TVecInitialFosterDiode=[25, 25] degC  no_thermal_network=ee.enum.enable.no  mosfet_junction_temperature_specify=off  mosfet_junction_temperature_priority=None  mosfet_junction_temperature=25 degC  mosfet_junction_temperature_nominal_specify=off  mosfet_junction_temperature_nominal_value=1  mosfet_junction_temperature_nominal_unit=degC  diode_junction_temperature_specify=off  diode_junction_temperature_priority=None  diode_junction_temperature=25 degC  diode_junction_temperature_nominal_specify=off  diode_junction_temperature_nominal_value=1  diode_junction_temperature_nominal_unit=degC  Qj_specify=off  Qj_priority=None  Qj=0 W  Qj_nominal_specify=off  Qj_nominal_value=1  Qj_nominal_unit=W  accumulatedSwitchingLosses_specify=off  accumulatedSwitchingLosses_priority=None  accumulatedSwitchingLosses=0 J
  Simulink-PS Converter : nesl_utility/Simulink-PS Converter  PhysicalDomain=network_engine_domain  SubClassName=ps_input  LeftPortType=input  RightPortType=output  PseudoPeriodic=off  Frequencies=[]  NoiseDistribution=none  NoiseParameters=[]  Unit=1  AffineConversion=off  FilteringAndDerivatives=provide  SimscapeFilterOrder=1  InputFilterTimeConstant=0.001  UdotUserProvided=0
  D : PMIOPort  Side=Left
  S : PMIOPort  Port=2  Side=Right
  wires:
  Data Type Conversion/1 -> Simulink-PS Converter/1
  g/1 -> Data Type Conversion/1
  connections:
  MOSFET/RConn1 -- D/RConn1
  Simulink-PS Converter/RConn1 -- MOSFET/LConn1
  S/RConn1 -- MOSFET/RConn2

== system DWPT_250k_60V/Synchronous Rectifier/Q3 ==
  g : Inport
  Data Type Conversion : DataTypeConversion  OutDataTypeStr=double  SaturateOnIntegerOverflow=off  RndMeth=Floor
  MOSFET : ee_lib/Semiconductors & Converters/MOSFET (Ideal, Switching)  port_option=ee.enum.controlport.ps  Rds=RonSR Ohm  Goff=Goff 1/Ohm  Vth=0.5 V  diode_param=2  diode_Vf=bodyVf V  diode_Ron=bodyRon Ohm  diode_Goff=Goff 1/Ohm  diode_C=5e-8 F  diode_iRM=-235 A  diode_iF=300 A  diode_idot=-50 A/us  diode_trr_param=1  diode_trr_factor=3  diode_trr=15 us  diode_Qrr=1.5e+3 s*uA  ids_specify=off  ids_priority=None  ids=0 A  ids_nominal_specify=off  ids_nominal_value=1  ids_nominal_unit=A  vds_specify=off  vds_priority=None  vds=0 V  vds_nominal_specify=off  vds_nominal_value=1  vds_nominal_unit=V  vgs_specify=off  vgs_priority=None  vgs=0 V  vgs_nominal_specify=off  vgs_nominal_value=1  vgs_nominal_unit=V  thermal_loss_option=ee.enum.converters.thermalLossOption.constantvalues  Von_data=[0, 1.1, 1.3, 1.45, 1.75, 2.25, 2.7; 0, 1, 1.15, 1.35, 1.7, 2.35, 3] V  Tj=[298.15, 398.15] K  Iout_data=[0, 10, 50, 100, 200, 400, 600] A  tabulateWithVds=false  Eon_data=[0, .29, 1.43, 2.86, 5.71, 13.14, 22.86; 0, .57, 2.63, 5.14, 10.29, 20.57, 30.29] * 1e-3 J  Eoff_data=[0, .21, 1.07, 2.14, 4.29, 9.86, 17.14; 0, .43, 1.97, 3.86, 7.71, 15.43, 22.71] * 1e-3 J  Eon_data_3D=[zeros(2, 5, 3)] J  Eoff_data_3D=[zeros(2, 5, 3)] J  Tj_loss=[298.15, 448.15] K  Iout_data_loss=[0, 10, 20, 30, 40] A  Vds_loss=[0, 150, 300] V  Eon_scalar=22.86e-3 J  Eoff_scalar=17.14e-3 J  Voff=300 V  Iout_scalar=600 A  useCurrentFromPreviousCycle=true  currentMeasDelay=0 s  useVoltageFromPreviousCycle=true  voltageMeasDelay=0 s  diodeModelType=ee.enum.converters.diodeModelType.pwl  diodeTableType=ee.enum.diode.tableType.IfMat  diode_ReverseIVType=ee.enum.diode.diodeReverseIV.constant  diode_IfMat=[.07, .12, .19, 1.75, 4.24, 7.32, 11.2; .16, .3, .72, 2.14, 4.02, 6.35, 9.12] A  diode_VfMat=[.9, 1.15, 1.25, 1.5, 1.75, 2.17, 2.6, 2.85; .58, .68, .75, 1.1, 1.38, 1.77, 2.27, 2.7] V  diode_TjVec=[25, 125] degC  diode_VfVec=[.5, .7, .9, 1.3, 1.7, 2.1, 2.5] V  diode_IfVec=[.1, .2, .5, 1, 2, 4, 7, 10] A  diode_IrMat=[1e-06, 2e-06, 5e-06, 1e-05, 2.5e-05, 5e-05, .0001; 2e-06, 5e-06, 1e-05, 4e-05, 8e-05, .0002, .0005] A  diode_VrMat=[10, 100, 200, 250, 300, 325, 350; 10, 70, 160, 220, 270, 300, 320] V  diode_VrVec=[10, 20, 40, 50, 70, 80, 100] V  diode_IrVec=[1e-06, 2e-06, 5e-06, 1e-05, 2e-05, 5e-05, .0001] A  diode_Vr=-600 V  diode_Ls=150 nH  diode_Erec=0.03 J  diode_rec_loss_model=ee.enum.diode.reverseRecoveryModelTabulateUpTo3D.fixed  diode_ErecVal=0 J  diode_scaleWithIandV=true  diode_ErecMat=zeros(2, 3) J  diodeErecMat3D=zeros(2, 3, 2) J  diode_TjrecVec=[298.15, 398.15] K  diode_IfrecVec=[.1, 1, 10] A  diodeVrecVec=[0, 100] V  diode_IrecVal=10 A  diode_VrecVal=10 V  diode_tFilter=1 / 1000 / 100 s  separateThermalPortForDiode=false  thermal_network_parameterization=ee.enum.thermalNetworkTopology.external  Rth=[.03, .2] K/W  Rth_Cauer=[.03, .1, .2] K/W  Rth_Foster=[.03, .2] K/W  thermal_mass_parameterization=ee.enum.thermalNetwork.timeconstant  thermal_mass=[3, 25] J/K  thermal_mass_Cauer=[3, 10, 25] J/K  thermal_mass_Foster=[33, 50] J/K  thermal_time_constant=[.1, 5] s  thermal_time_constant_Cauer=[.1, 1, 5] s  thermal_time_constant_Foster=[1, 10] s  thermal_mass_initial_temperatures=[25, 25] degC  thermal_mass_initial_temperatures_Cauer=[25, 25, 25] degC  junction_thermal_mass=0.1 J/K  Tvec_initial_Foster=[25, 25, 25, 25] degC  RthDiode=[.03, .2] K/W  RthCauerDiode=[.03, .1, .2] K/W  RthFosterDiode=[.03, .2] K/W  thermalMassDiode=[3, 25] J/K  thermalMassCauerDiode=[3, 10, 25] J/K  thermalMassFosterDiode=[33, 50] J/K  thermalTauDiode=[.1, 5] s  thermalTauCauerDiode=[.1, 1, 5] s  thermalTauFosterDiode=[1, 10] s  thermalMassInitTempDiode=[25, 25] degC  thermalMassInitTempCauerDiode=[25, 25, 25] degC  junctionthermalMassDiode=0.1 J/K  TVecInitialFosterDiode=[25, 25] degC  no_thermal_network=ee.enum.enable.no  mosfet_junction_temperature_specify=off  mosfet_junction_temperature_priority=None  mosfet_junction_temperature=25 degC  mosfet_junction_temperature_nominal_specify=off  mosfet_junction_temperature_nominal_value=1  mosfet_junction_temperature_nominal_unit=degC  diode_junction_temperature_specify=off  diode_junction_temperature_priority=None  diode_junction_temperature=25 degC  diode_junction_temperature_nominal_specify=off  diode_junction_temperature_nominal_value=1  diode_junction_temperature_nominal_unit=degC  Qj_specify=off  Qj_priority=None  Qj=0 W  Qj_nominal_specify=off  Qj_nominal_value=1  Qj_nominal_unit=W  accumulatedSwitchingLosses_specify=off  accumulatedSwitchingLosses_priority=None  accumulatedSwitchingLosses=0 J
  Simulink-PS Converter : nesl_utility/Simulink-PS Converter  PhysicalDomain=network_engine_domain  SubClassName=ps_input  LeftPortType=input  RightPortType=output  PseudoPeriodic=off  Frequencies=[]  NoiseDistribution=none  NoiseParameters=[]  Unit=1  AffineConversion=off  FilteringAndDerivatives=provide  SimscapeFilterOrder=1  InputFilterTimeConstant=0.001  UdotUserProvided=0
  D : PMIOPort  Side=Left
  S : PMIOPort  Port=2  Side=Right
  wires:
  Data Type Conversion/1 -> Simulink-PS Converter/1
  g/1 -> Data Type Conversion/1
  connections:
  MOSFET/RConn1 -- D/RConn1
  Simulink-PS Converter/RConn1 -- MOSFET/LConn1
  S/RConn1 -- MOSFET/RConn2

== system DWPT_250k_60V/Synchronous Rectifier/Q4 ==
  g : Inport
  Data Type Conversion : DataTypeConversion  OutDataTypeStr=double  SaturateOnIntegerOverflow=off  RndMeth=Floor
  MOSFET : ee_lib/Semiconductors & Converters/MOSFET (Ideal, Switching)  port_option=ee.enum.controlport.ps  Rds=RonSR Ohm  Goff=Goff 1/Ohm  Vth=0.5 V  diode_param=2  diode_Vf=bodyVf V  diode_Ron=bodyRon Ohm  diode_Goff=Goff 1/Ohm  diode_C=5e-8 F  diode_iRM=-235 A  diode_iF=300 A  diode_idot=-50 A/us  diode_trr_param=1  diode_trr_factor=3  diode_trr=15 us  diode_Qrr=1.5e+3 s*uA  ids_specify=off  ids_priority=None  ids=0 A  ids_nominal_specify=off  ids_nominal_value=1  ids_nominal_unit=A  vds_specify=off  vds_priority=None  vds=0 V  vds_nominal_specify=off  vds_nominal_value=1  vds_nominal_unit=V  vgs_specify=off  vgs_priority=None  vgs=0 V  vgs_nominal_specify=off  vgs_nominal_value=1  vgs_nominal_unit=V  thermal_loss_option=ee.enum.converters.thermalLossOption.constantvalues  Von_data=[0, 1.1, 1.3, 1.45, 1.75, 2.25, 2.7; 0, 1, 1.15, 1.35, 1.7, 2.35, 3] V  Tj=[298.15, 398.15] K  Iout_data=[0, 10, 50, 100, 200, 400, 600] A  tabulateWithVds=false  Eon_data=[0, .29, 1.43, 2.86, 5.71, 13.14, 22.86; 0, .57, 2.63, 5.14, 10.29, 20.57, 30.29] * 1e-3 J  Eoff_data=[0, .21, 1.07, 2.14, 4.29, 9.86, 17.14; 0, .43, 1.97, 3.86, 7.71, 15.43, 22.71] * 1e-3 J  Eon_data_3D=[zeros(2, 5, 3)] J  Eoff_data_3D=[zeros(2, 5, 3)] J  Tj_loss=[298.15, 448.15] K  Iout_data_loss=[0, 10, 20, 30, 40] A  Vds_loss=[0, 150, 300] V  Eon_scalar=22.86e-3 J  Eoff_scalar=17.14e-3 J  Voff=300 V  Iout_scalar=600 A  useCurrentFromPreviousCycle=true  currentMeasDelay=0 s  useVoltageFromPreviousCycle=true  voltageMeasDelay=0 s  diodeModelType=ee.enum.converters.diodeModelType.pwl  diodeTableType=ee.enum.diode.tableType.IfMat  diode_ReverseIVType=ee.enum.diode.diodeReverseIV.constant  diode_IfMat=[.07, .12, .19, 1.75, 4.24, 7.32, 11.2; .16, .3, .72, 2.14, 4.02, 6.35, 9.12] A  diode_VfMat=[.9, 1.15, 1.25, 1.5, 1.75, 2.17, 2.6, 2.85; .58, .68, .75, 1.1, 1.38, 1.77, 2.27, 2.7] V  diode_TjVec=[25, 125] degC  diode_VfVec=[.5, .7, .9, 1.3, 1.7, 2.1, 2.5] V  diode_IfVec=[.1, .2, .5, 1, 2, 4, 7, 10] A  diode_IrMat=[1e-06, 2e-06, 5e-06, 1e-05, 2.5e-05, 5e-05, .0001; 2e-06, 5e-06, 1e-05, 4e-05, 8e-05, .0002, .0005] A  diode_VrMat=[10, 100, 200, 250, 300, 325, 350; 10, 70, 160, 220, 270, 300, 320] V  diode_VrVec=[10, 20, 40, 50, 70, 80, 100] V  diode_IrVec=[1e-06, 2e-06, 5e-06, 1e-05, 2e-05, 5e-05, .0001] A  diode_Vr=-600 V  diode_Ls=150 nH  diode_Erec=0.03 J  diode_rec_loss_model=ee.enum.diode.reverseRecoveryModelTabulateUpTo3D.fixed  diode_ErecVal=0 J  diode_scaleWithIandV=true  diode_ErecMat=zeros(2, 3) J  diodeErecMat3D=zeros(2, 3, 2) J  diode_TjrecVec=[298.15, 398.15] K  diode_IfrecVec=[.1, 1, 10] A  diodeVrecVec=[0, 100] V  diode_IrecVal=10 A  diode_VrecVal=10 V  diode_tFilter=1 / 1000 / 100 s  separateThermalPortForDiode=false  thermal_network_parameterization=ee.enum.thermalNetworkTopology.external  Rth=[.03, .2] K/W  Rth_Cauer=[.03, .1, .2] K/W  Rth_Foster=[.03, .2] K/W  thermal_mass_parameterization=ee.enum.thermalNetwork.timeconstant  thermal_mass=[3, 25] J/K  thermal_mass_Cauer=[3, 10, 25] J/K  thermal_mass_Foster=[33, 50] J/K  thermal_time_constant=[.1, 5] s  thermal_time_constant_Cauer=[.1, 1, 5] s  thermal_time_constant_Foster=[1, 10] s  thermal_mass_initial_temperatures=[25, 25] degC  thermal_mass_initial_temperatures_Cauer=[25, 25, 25] degC  junction_thermal_mass=0.1 J/K  Tvec_initial_Foster=[25, 25, 25, 25] degC  RthDiode=[.03, .2] K/W  RthCauerDiode=[.03, .1, .2] K/W  RthFosterDiode=[.03, .2] K/W  thermalMassDiode=[3, 25] J/K  thermalMassCauerDiode=[3, 10, 25] J/K  thermalMassFosterDiode=[33, 50] J/K  thermalTauDiode=[.1, 5] s  thermalTauCauerDiode=[.1, 1, 5] s  thermalTauFosterDiode=[1, 10] s  thermalMassInitTempDiode=[25, 25] degC  thermalMassInitTempCauerDiode=[25, 25, 25] degC  junctionthermalMassDiode=0.1 J/K  TVecInitialFosterDiode=[25, 25] degC  no_thermal_network=ee.enum.enable.no  mosfet_junction_temperature_specify=off  mosfet_junction_temperature_priority=None  mosfet_junction_temperature=25 degC  mosfet_junction_temperature_nominal_specify=off  mosfet_junction_temperature_nominal_value=1  mosfet_junction_temperature_nominal_unit=degC  diode_junction_temperature_specify=off  diode_junction_temperature_priority=None  diode_junction_temperature=25 degC  diode_junction_temperature_nominal_specify=off  diode_junction_temperature_nominal_value=1  diode_junction_temperature_nominal_unit=degC  Qj_specify=off  Qj_priority=None  Qj=0 W  Qj_nominal_specify=off  Qj_nominal_value=1  Qj_nominal_unit=W  accumulatedSwitchingLosses_specify=off  accumulatedSwitchingLosses_priority=None  accumulatedSwitchingLosses=0 J
  Simulink-PS Converter : nesl_utility/Simulink-PS Converter  PhysicalDomain=network_engine_domain  SubClassName=ps_input  LeftPortType=input  RightPortType=output  PseudoPeriodic=off  Frequencies=[]  NoiseDistribution=none  NoiseParameters=[]  Unit=1  AffineConversion=off  FilteringAndDerivatives=provide  SimscapeFilterOrder=1  InputFilterTimeConstant=0.001  UdotUserProvided=0
  D : PMIOPort  Side=Left
  S : PMIOPort  Port=2  Side=Right
  wires:
  Data Type Conversion/1 -> Simulink-PS Converter/1
  g/1 -> Data Type Conversion/1
  connections:
  MOSFET/RConn1 -- D/RConn1
  Simulink-PS Converter/RConn1 -- MOSFET/LConn1
  S/RConn1 -- MOSFET/RConn2
